simulink model "ex_01_sim"  (R2024b)
settings: Solver=VariableStepAuto  StartTime=0.0  StopTime=10.0  RelTol=1e-3
values from neighbouring files (symbols this model uses):
  A = d.A    [ex_01_main.m]
  B = d.B    [ex_01_main.m]
  C = d.C    [ex_01_main.m]
  D = d.D    [ex_01_main.m]
undefined symbols (not defined in the file or in its folder): K
settings Model: Creator=54238  LastModifiedBy=54238

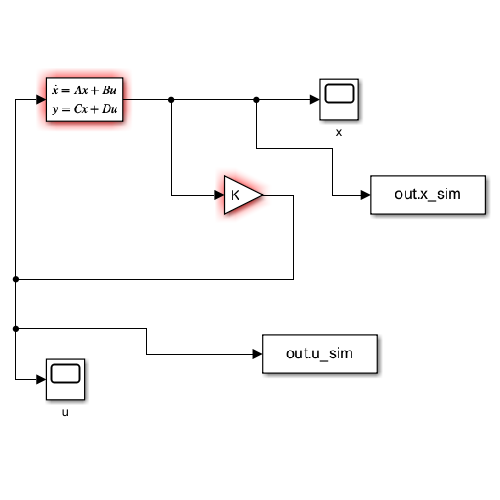
[thumbnail: Simulink's stored preview of the top-level diagram]
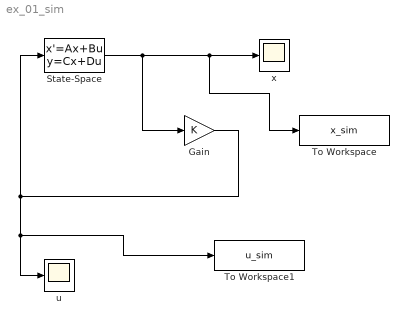
== system ex_01_sim ==
  Gain : Gain  Gain=K
  State-Space : StateSpace  A=A  B=B  C=C  D=D  InitialCondition=0
  To Workspace : ToWorkspace  VariableName=x_sim  SaveFormat=Timeseries  SampleTime=-1
  To Workspace1 : ToWorkspace  VariableName=u_sim  SaveFormat=Timeseries  SampleTime=-1
  u : Scope
  x : Scope
  wires:
  State-Space/1 -> To Workspace/1, x/1, Gain/1
  Gain/1 -> State-Space/1, To Workspace1/1, u/1
